simulink model "QDVoltageTunableDownconverter"  (R2026a)
settings: Solver=FixedStepDiscrete  StartTime=0  StopTime=0  FixedStep=1
InitFcn:
  | initQDVoltageTunableDualConverter(false);
undefined symbols (not defined in the file or in its folder): qdCommonOutputWavelength_nm, qdInGaAsDetectorGain_ePerPhoton, qdSiDetectorGain_ePerPhoton, qdUVIncidentSpectrum
Description:
  | Passive UV-to-visible/NIR QD film bank selected by an electronic voltage decoder, split silicon/InGaAs detection, and UV spectral reconstruction from spatial filter measurements.
settings Model: Creator=jyohtiprakash  LastModifiedBy=jyohtiprakash

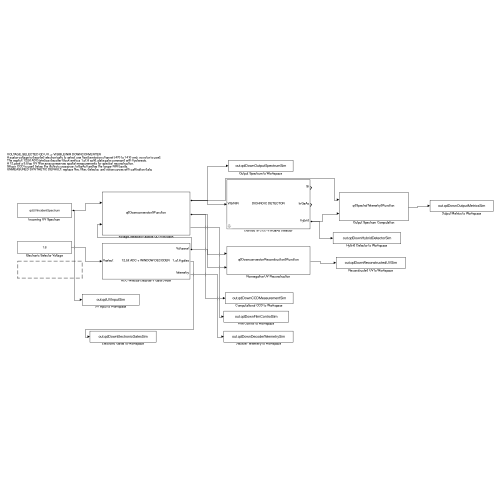
[thumbnail: Simulink's stored preview of the top-level diagram]
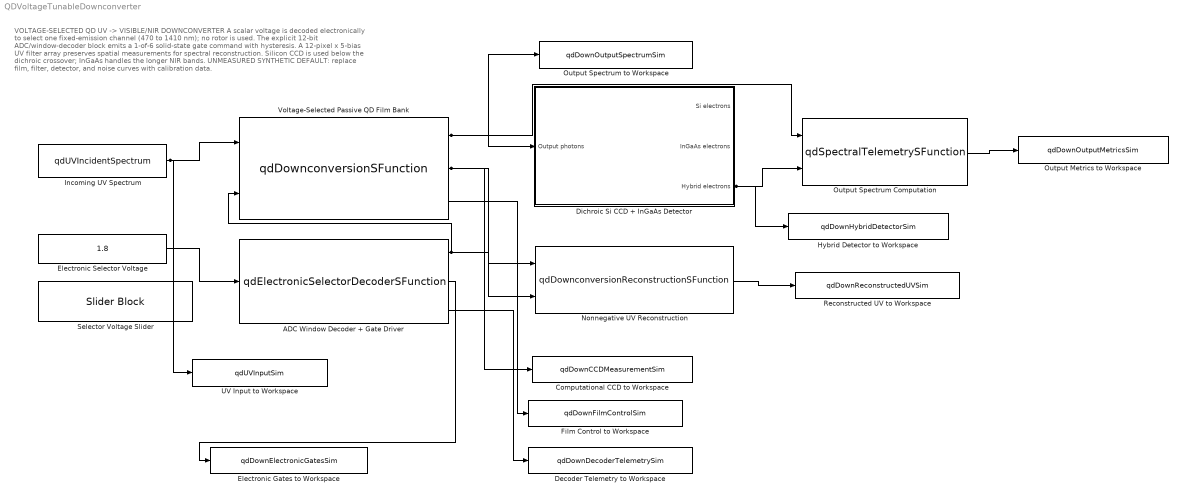
== system QDVoltageTunableDownconverter ==
  note: VOLTAGE-SELECTED QD UV -> VISIBLE/NIR DOWNCONVERTER
      | A scalar voltage is decoded electronically to select one fixed-emission channel (470 to 1410 nm); no rotor is used.
      | The explicit 12-bit ADC/window-decoder block emits a 1-of-6 solid-state gate command with hysteresis.
      | A 12-pixel x 5-bias UV filter array preserves spatial measurements for spectral reconstruction.
      | Silicon CCD is used below the dichroic crossover; InGaAs handles the longer NIR bands.
      | UNMEASURED SYNTHETIC DEFAULT: replace film, filter, detector, and noise curves with calibration data.
  ADC Window Decoder + Gate Driver : M-S-Function  FunctionName=qdElectronicSelectorDecoderSFunction
      mask help: Electronic selector: ADC quantization, voltage-window decoding, comparator hysteresis, and one-hot optical-gate command.
      mask Display:
      | disp('12-bit ADC + WINDOW DECODER');
      | port_label('input',1,'Vselect');
      | port_label('output',1,'Vchannel');
      | port_label('output',2,'1-of-6 gates');
      | port_label('output',3,'telemetry');
  Computational CCD to Workspace : ToWorkspace  VariableName=qdDownCCDMeasurementSim  SaveFormat=Structure With Time  SampleTime=-1
  Decoder Telemetry to Workspace : ToWorkspace  VariableName=qdDownDecoderTelemetrySim  SaveFormat=Structure With Time  SampleTime=-1
  Dichroic Si CCD + InGaAs Detector : Subsystem
      mask help: Dichroic split detector: silicon CCD for visible/NIR-I and InGaAs for wavelengths beyond the silicon cutoff.
      mask Display:
      | disp('DICHROIC DETECTOR');
      | port_label('input',1,'VIS/NIR');
      | port_label('output',1,'Si');
      | port_label('output',2,'InGaAs');
      | port_label('output',3,'hybrid');
  Electronic Gates to Workspace : ToWorkspace  VariableName=qdDownElectronicGatesSim  SaveFormat=Structure With Time  SampleTime=-1
  Electronic Selector Voltage : Constant  Value=1.8
  Film Control to Workspace : ToWorkspace  VariableName=qdDownFilmControlSim  SaveFormat=Structure With Time  SampleTime=-1
  Hybrid Detector to Workspace : ToWorkspace  VariableName=qdDownHybridDetectorSim  SaveFormat=Structure With Time  SampleTime=-1
  Incoming UV Spectrum : Constant  Value=qdUVIncidentSpectrum
  Nonnegative UV Reconstruction : M-S-Function  FunctionName=qdDownconversionReconstructionSFunction
  Output Metrics to Workspace : ToWorkspace  VariableName=qdDownOutputMetricsSim  SaveFormat=Structure With Time  SampleTime=-1
  Output Spectrum Computation : M-S-Function  FunctionName=qdSpectralTelemetrySFunction
  Output Spectrum to Workspace : ToWorkspace  VariableName=qdDownOutputSpectrumSim  SaveFormat=Structure With Time  SampleTime=-1
  Reconstructed UV to Workspace : ToWorkspace  VariableName=qdDownReconstructedUVSim  SaveFormat=Structure With Time  SampleTime=-1
  Selector Voltage Slider : SliderBlock  ScaleMin=0.29999999999999999  ScaleMax=2.7999999999999998  TickInterval=0.49999999999999978
  UV Input to Workspace : ToWorkspace  VariableName=qdUVInputSim  SaveFormat=Structure With Time  SampleTime=-1
  Voltage-Selected Passive QD Film Bank : M-S-Function  FunctionName=qdDownconversionSFunction
  wires:
  Electronic Selector Voltage/1 -> ADC Window Decoder + Gate Driver/1
  Incoming UV Spectrum/1 -> Voltage-Selected Passive QD Film Bank/1, UV Input to Workspace/1
  ADC Window Decoder + Gate Driver/1 -> Voltage-Selected Passive QD Film Bank/2, Nonnegative UV Reconstruction/2
  Voltage-Selected Passive QD Film Bank/1 -> Dichroic Si CCD + InGaAs Detector/1(Output photons), Output Spectrum Computation/1, Output Spectrum to Workspace/1
  Voltage-Selected Passive QD Film Bank/2 -> Nonnegative UV Reconstruction/1, Computational CCD to Workspace/1
  Dichroic Si CCD + InGaAs Detector/3(Hybrid electrons) -> Output Spectrum Computation/2, Hybrid Detector to Workspace/1
  Voltage-Selected Passive QD Film Bank/3 -> Film Control to Workspace/1
  ADC Window Decoder + Gate Driver/2 -> Electronic Gates to Workspace/1
  ADC Window Decoder + Gate Driver/3 -> Decoder Telemetry to Workspace/1
  Nonnegative UV Reconstruction/1 -> Reconstructed UV to Workspace/1
  Output Spectrum Computation/1 -> Output Metrics to Workspace/1

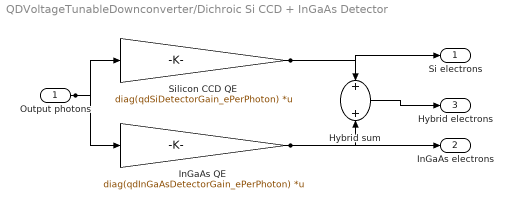
== system QDVoltageTunableDownconverter/Dichroic Si CCD + InGaAs Detector ==
  Output photons : Inport  PortDimensions=numel(qdCommonOutputWavelength_nm)
  Hybrid sum : Sum
  InGaAs QE : Gain  Gain=diag(qdInGaAsDetectorGain_ePerPhoton)  Multiplication=Matrix(K*u)
  Silicon CCD QE : Gain  Gain=diag(qdSiDetectorGain_ePerPhoton)  Multiplication=Matrix(K*u)
  Si electrons : Outport  PortDimensions=numel(qdCommonOutputWavelength_nm)
  InGaAs electrons : Outport  Port=2  PortDimensions=numel(qdCommonOutputWavelength_nm)
  Hybrid electrons : Outport  Port=3  PortDimensions=numel(qdCommonOutputWavelength_nm)
  wires:
  Output photons/1 -> Silicon CCD QE/1, InGaAs QE/1
  Silicon CCD QE/1 -> Hybrid sum/1, Si electrons/1
  InGaAs QE/1 -> Hybrid sum/2, InGaAs electrons/1
  Hybrid sum/1 -> Hybrid electrons/1
